simulink model "schemat"  (R2026b)
settings: Solver=VariableStepAuto
values from neighbouring files (symbols this model uses):
  cpro = cp * rop    (= 1200)    [script.m]
  Cv1 = cpro * A1 * h    (= 100000)    [script.m]
  Cv2 = cpro * A2 * h    (= 50000)    [script.m]
  dfp = skoki(j, 3)    [script.m]
  dTkz = skoki(j, 1)    [script.m]
  dTzew = skoki(j, 2)    [script.m]
  fp_0 = tab_Fp(i)    [script.m]
  K0 = (PkN - Ks1 * (Tw1N - TzewN)) / (Tw1N - Tw2N)    (= 608.695652174)    [script.m]
  Ks1 = a * Ks2    (= 173.913043478)    [script.m]
  Ks2 = PkN / (a * (Tw1N - TzewN) + (Tw2N - TzewN))    (= 86.9565217391)    [script.m]
  t_skok = 200    [script.m]
  Tkz_0 = tab_Tkz(i)    [script.m]
  Tw1_0 = tab_Tw1(i)    [script.m]
  Tw2_0 = tab_Tw2(i)    [script.m]
  Tzew_0 = tab_Tzew(i)    [script.m]
settings Model: Creator=marcel  LastModifiedBy=marcel

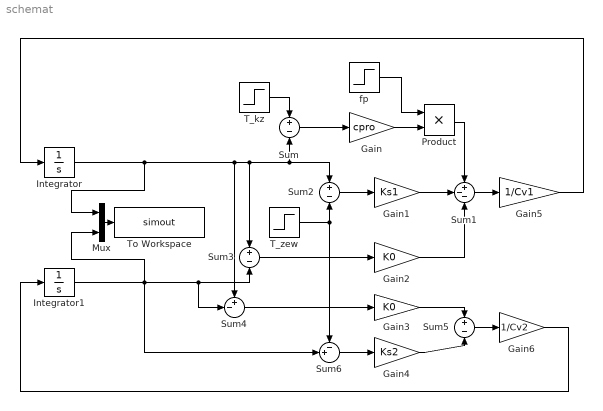
== system schemat ==
  Gain : Gain  Gain=cpro
  Gain1 : Gain  Gain=Ks1
  Gain2 : Gain  Gain=K0
  Gain3 : Gain  Gain=K0
  Gain4 : Gain  Gain=Ks2
  Gain5 : Gain  Gain=1/Cv1
  Gain6 : Gain  Gain=1/Cv2
  Integrator : Integrator  InitialCondition=Tw1_0
  Integrator1 : Integrator  InitialCondition=Tw2_0
  Mux : Mux  Inputs=2
  Product : Product
  Sum{,2..3,5} (4 alike) : Sum  Inputs=+-
  Sum1 : Sum  Inputs=+--
  Sum4 : Sum  Inputs=+-|
  Sum6 : Sum  Inputs=-+|
  T_kz : Step  Time=t_skok  InitialValue=Tkz_0  FinalValue=Tkz_0 + dTkz  SampleTime=0
  T_zew : Step  Time=t_skok  InitialValue=Tzew_0  FinalValue=Tzew_0 + dTzew  SampleTime=0
  To Workspace : ToWorkspace  VariableName=simout  SaveFormat=Timeseries  SampleTime=-1
  fp : Step  Time=t_skok  InitialValue=fp_0  FinalValue=fp_0 + dfp  SampleTime=0
  wires:
  Integrator/1 -> Sum4/1, Sum3/1, Sum2/1, Sum/2, Mux/1
  Integrator1/1 -> Sum6/2, Sum4/2, Sum3/2, Mux/2
  T_kz/1 -> Sum/1
  Sum2/1 -> Gain1/1
  Gain1/1 -> Sum1/2
  T_zew/1 -> Sum6/1, Sum2/2
  Sum3/1 -> Gain2/1
  Gain2/1 -> Sum1/3
  Sum4/1 -> Gain3/1
  Gain3/1 -> Sum5/1
  Sum6/1 -> Gain4/1
  Gain4/1 -> Sum5/2
  Mux/1 -> To Workspace/1
  Sum1/1 -> Gain5/1
  Sum5/1 -> Gain6/1
  Gain5/1 -> Integrator/1
  Gain6/1 -> Integrator1/1
  Product/1 -> Sum1/1
  fp/1 -> Product/1
  Sum/1 -> Gain/1
  Gain/1 -> Product/2
